simulink model "closedloopDAB"  (R2024b)
settings: Solver=ode23t  StartTime=0.0  StopTime=0.01  FixedStep=Tsolver  MaxStep=Tsolver  RelTol=1e-05
values from neighbouring files (symbols this model uses):
  D1 = M.D(k,1)    [closedloop_init.m]    (also in validate_exact_model.m)
  D2 = M.D(k,2)    [closedloop_init.m]    (also in validate_exact_model.m)
  D3 = M.D(k,3)    [closedloop_init.m]    (also in validate_exact_model.m)
  f_sw = P.fs    [closedloop_init.m]    (also in validate_exact_model.m)
  i2_cmd_max = umax_cmd    [closedloop_init.m]
  i2_cmd_min = -umax_cmd    [closedloop_init.m]
  Iref0 = -41.3    [closedloop_init.m]
  Iref1 = -46.3    [closedloop_init.m]
  ki_cmd = -5.2995    [closedloop_init.m]
  kp_cmd = -5.2995e-05    [closedloop_init.m]
  Ri = P.R1    [closedloop_init.m]    (also in validate_exact_model.m)
  Ro = P.R2    [closedloop_init.m]    (also in validate_exact_model.m)
  Rs = P.R    [closedloop_init.m]    (also in validate_exact_model.m)
  t_step = 5e-3    (= 0.005)    [closedloop_init.m]
  tdead = 0    [closedloop_init.m]    (also in validate_exact_model.m)
  umax_cmd = 0.8*min(D3 - 0, (D1 - D2) - D3)    [closedloop_init.m]
  Vi = P.V1    [closedloop_init.m]    (also in validate_exact_model.m)
  Vo = P.V2    [closedloop_init.m]    (also in validate_exact_model.m)
  Vth = 0.5    [closedloop_init.m]    (also in validate_exact_model.m)
libraries: fl_lib x15, nesl_utility x13, ee_lib x8, slpidlib x1, simulink x1
settings Model: Creator=amina  LastModifiedBy=amina
settings DataIOCC: SaveOutput=off  SignalLogging=off  DSMLogging=off  SaveTime=off  ReturnWorkspaceOutputs=off  ReturnWorkspaceOutputsName=out_fwd

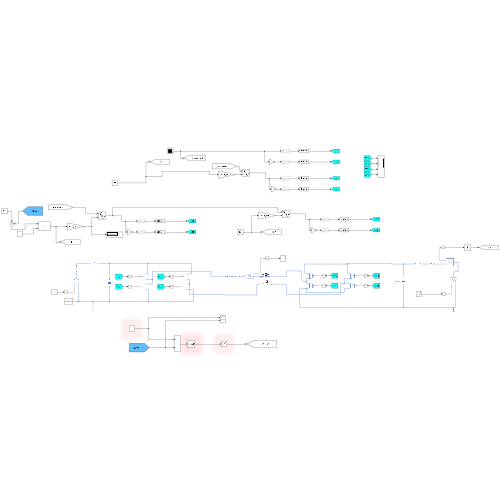
[thumbnail: Simulink's stored preview of the top-level diagram]
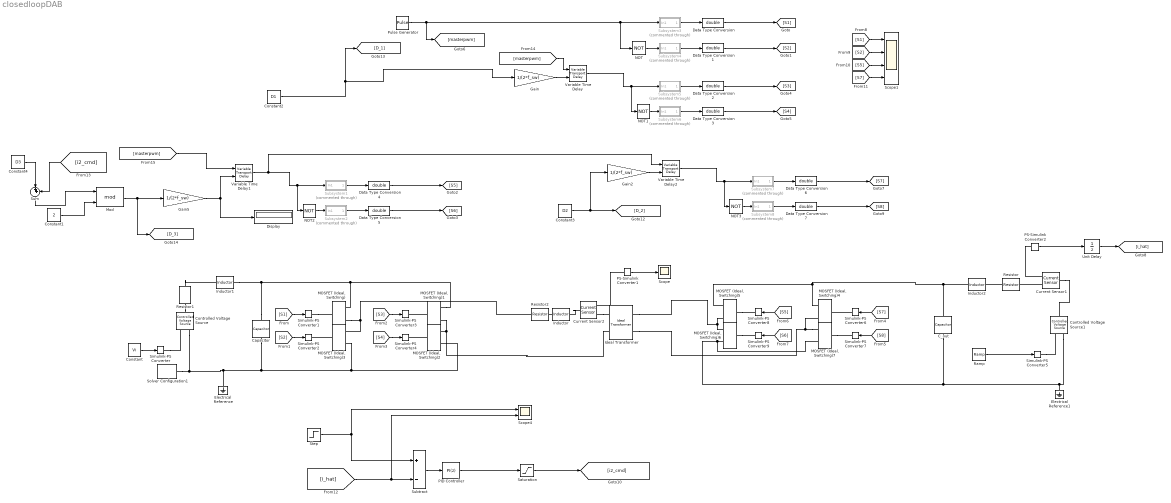
== system closedloopDAB ==
  C_out : fl_lib/Electrical/Electrical Elements/Capacitor  c=Co F  r=0 Ohm  g=0 1/Ohm  i_specify=off  i_priority=None  i=0 A  i_nominal_specify=off  i_nominal_value=1  i_nominal_unit=A  v_specify=off  v_priority=None  v=0 V  v_nominal_specify=off  v_nominal_value=1  v_nominal_unit=V  vc_specify=off  vc_priority=High  vc=V_cap_init V  vc_nominal_specify=off  vc_nominal_value=1  vc_nominal_unit=V
  Capacitor : fl_lib/Electrical/Electrical Elements/Capacitor  c=Ci F  r=1e-6 Ohm  g=0 1/Ohm  i_specify=off  i_priority=None  i=0 A  i_nominal_specify=off  i_nominal_value=1  i_nominal_unit=A  v_specify=off  v_priority=None  v=0 V  v_nominal_specify=off  v_nominal_value=1  v_nominal_unit=V  vc_specify=off  vc_priority=High  vc=V_cap_init V  vc_nominal_specify=off  vc_nominal_value=1  vc_nominal_unit=V
  Constant : Constant  Value=Vi
  Constant1 : Constant  Value=2
  Constant2 : Constant  Value=D1
  Constant3 : Constant  Value=D2
  Constant4 : Constant  Value=D3
  Controlled Voltage Source : fl_lib/Electrical/Electrical Sources/Controlled Voltage Source
  Controlled Voltage Source1 : fl_lib/Electrical/Electrical Sources/Controlled Voltage Source
  Current Sensor1 : fl_lib/Electrical/Electrical Sensors/Current Sensor
  Current Sensor2 : fl_lib/Electrical/Electrical Sensors/Current Sensor
  Data Type Conversion{,1..7} (8 alike) : DataTypeConversion  OutDataTypeStr=double  SaturateOnIntegerOverflow=off  RndMeth=Floor
  Display : Display
  Electrical Reference : fl_lib/Electrical/Electrical Elements/Electrical Reference
  Electrical Reference1 : fl_lib/Electrical/Electrical Elements/Electrical Reference
  Gain : Gain  Gain=1/(2*f_sw)
  Gain2 : Gain  Gain=1/(2*f_sw)
  Gain5 : Gain  Gain=1/(2*f_sw)
  Ideal Transformer : fl_lib/Electrical/Electrical Elements/Ideal Transformer  n=n  i1_specify=off  i1_priority=None  i1=0 A  i1_nominal_specify=off  i1_nominal_value=1  i1_nominal_unit=A  v1_specify=off  v1_priority=None  v1=0 V  v1_nominal_specify=off  v1_nominal_value=1  v1_nominal_unit=V  i2_specify=off  i2_priority=None  i2=0 A  i2_nominal_specify=off  i2_nominal_value=1  i2_nominal_unit=A  v2_specify=off  v2_priority=None  v2=0 V  v2_nominal_specify=off  v2_nominal_value=1  v2_nominal_unit=V
  Inductor : fl_lib/Electrical/Electrical Elements/Inductor  l=Ls H  r=0 Ohm  g=1e-9 1/Ohm  i_specify=off  i_priority=None  i=0 A  i_nominal_specify=off  i_nominal_value=1  i_nominal_unit=A  v_specify=off  v_priority=None  v=0 V  v_nominal_specify=off  v_nominal_value=1  v_nominal_unit=V  i_L_specify=off  i_L_priority=High  i_L=0 A  i_L_nominal_specify=off  i_L_nominal_value=1  i_L_nominal_unit=A
  Inductor1 : fl_lib/Electrical/Electrical Elements/Inductor  l=Li H  r=0 Ohm  g=1e-9 1/Ohm  i_specify=off  i_priority=None  i=0 A  i_nominal_specify=off  i_nominal_value=1  i_nominal_unit=A  v_specify=off  v_priority=None  v=0 V  v_nominal_specify=off  v_nominal_value=1  v_nominal_unit=V  i_L_specify=off  i_L_priority=High  i_L=0 A  i_L_nominal_specify=off  i_L_nominal_value=1  i_L_nominal_unit=A
  Inductor2 : fl_lib/Electrical/Electrical Elements/Inductor  l=Lo H  r=0 Ohm  g=1e-9 1/Ohm  i_specify=off  i_priority=None  i=0 A  i_nominal_specify=off  i_nominal_value=1  i_nominal_unit=A  v_specify=off  v_priority=None  v=0 V  v_nominal_specify=off  v_nominal_value=1  v_nominal_unit=V  i_L_specify=off  i_L_priority=High  i_L=0 A  i_L_nominal_specify=off  i_L_nominal_value=1  i_L_nominal_unit=A
  MOSFET (Ideal, Switching){,1..7} (8 alike) : ee_lib/Semiconductors & Converters/MOSFET (Ideal, Switching)  port_option=ee.enum.controlport.ps  Rds=Rds Ohm  Goff=G_mosfet 1/Ohm  Vth=Vth V  diode_param=ee.enum.semiconductors.protectionDiode.nodynamics  diode_Vf=0.8 V  diode_Ron=0.001 Ohm  diode_Goff=1e-5 1/Ohm  diode_C=50e-9 F  diode_iRM=-235 A  diode_iF=300 A  diode_idot=-50 A/us  diode_trr_param=ee.enum.converters.diodeReverseParam.trr_factor  diode_trr_factor=3  diode_trr=15 us  diode_Qrr=1500 s*uA  ids_specify=off  ids_priority=None  ids=0 A  ids_nominal_specify=off  ids_nominal_value=1  ids_nominal_unit=A  vds_specify=off  vds_priority=None  vds=0 V  vds_nominal_specify=off  vds_nominal_value=1  vds_nominal_unit=V  vgs_specify=off  vgs_priority=None  vgs=0 V  vgs_nominal_specify=off  vgs_nominal_value=1  vgs_nominal_unit=V  thermal_loss_option=ee.enum.converters.thermalLossOption.constantvalues  Von_data=[0, 1.8, 3.2, 6, 10, 16; 0, 2, 5.5, 9.5, 15, 25] V  Tj=[298.15, 448.15] K  Iout_data=[0, 20, 40, 60, 80, 100] A  Eon_data=[0, 55.04, 124.57, 235.53, 362.12; 0, 71.25, 161.25, 304.88, 468.75] * 1e-6 J  Eoff_data=[0, 18, 30, 56.1, 76.5; 0, 22.5, 37.5, 70.13, 95.63] * 1e-6 J  Eon_data_3D=[zeros(2, 5, 3)] J  Eoff_data_3D=[zeros(2, 5, 3)] J  Tj_loss=[298.15, 448.15] K  Iout_data_loss=[0, 10, 20, 30, 40] A  tabulateWithVds=false  Vds_loss=[0, 150, 300] V  Eon_scalar=22.86e-3 J  Eoff_scalar=17.14e-3 J  Voff=300 V  Iout_scalar=600 A  useCurrentFromPreviousCycle=false  useVoltageFromPreviousCycle=false  diodeModelType=ee.enum.converters.diodeModelType.pwl  diodeTableType=ee.enum.diode.tableType.IfMat  diode_ReverseIVType=ee.enum.diode.diodeReverseIV.constant  diode_IfMat=[.07, .12, .19, 1.75, 4.24, 7.32, 11.2; .16, .3, .72, 2.14, 4.02, 6.35, 9.12] A  diode_VfMat=[.9, 1.15, 1.25, 1.5, 1.75, 2.17, 2.6, 2.85; .58, .68, .75, 1.1, 1.38, 1.77, 2.27, 2.7] V  diode_TjVec=[25, 125] degC  diode_VfVec=[.5, .7, .9, 1.3, 1.7, 2.1, 2.5] V  diode_IfVec=[.1, .2, .5, 1, 2, 4, 7, 10] A  diode_IrMat=[1e-06, 2e-06, 5e-06, 1e-05, 2.5e-05, 5e-05, .0001; 2e-06, 5e-06, 1e-05, 4e-05, 8e-05, .0002, .0005] A  diode_VrMat=[10, 100, 200, 250, 300, 325, 350; 10, 70, 160, 220, 270, 300, 320] V  diode_VrVec=[10, 20, 40, 50, 70, 80, 100] V  diode_IrVec=[1e-06, 2e-06, 5e-06, 1e-05, 2e-05, 5e-05, .0001] A  diode_Vr=-600 V  diode_Ls=150 nH  diode_Erec=0.03 J  diode_rec_loss_model=ee.enum.diode.reverseRecoveryModel.fixed  diode_ErecVal=0 J  diode_scaleWithIandV=true  diode_ErecMat=zeros(2, 3) J  diode_TjrecVec=[298.15, 398.15] K  diode_IfrecVec=[.1, 1, 10] A  diode_IrecVal=10 A  diode_VrecVal=10 V  diode_tFilter=1 / 1000 / 100 s  separateThermalPortForDiode=false  thermal_network_parameterization=ee.enum.thermalNetworkTopology.external  Rth=[.03, .2] K/W  Rth_Cauer=[.03, .1, .2] K/W  Rth_Foster=[.08, .14, .22, .16] K/W  thermal_mass_parameterization=ee.enum.thermalNetwork.timeconstant  thermal_mass=[3, 25] J/K  thermal_mass_Cauer=[3, 10, 25] J/K  thermal_mass_Foster=[.001, .005, .05, .5] J/K  thermal_time_constant=[.1, 5] s  thermal_time_constant_Cauer=[.1, 1, 5] s  thermal_time_constant_Foster=[7e-05, .0007, .01, .08] s  thermal_mass_initial_temperatures=[25, 25] degC  thermal_mass_initial_temperatures_Cauer=[25, 25, 25] degC  junction_thermal_mass=0.1 J/K  Tvec_initial_Foster=[25, 25, 25, 25] degC  RthDiode=[.03, .2] K/W  RthCauerDiode=[.03, .1, .2] K/W  RthFosterDiode=[.03, .2] K/W  thermalMassDiode=[3, 25] J/K  thermalMassCauerDiode=[3, 10, 25] J/K  thermalMassFosterDiode=[33, 50] J/K  thermalTauDiode=[.1, 5] s  thermalTauCauerDiode=[.1, 1, 5] s  thermalTauFosterDiode=[1, 10] s  thermalMassInitTempDiode=[25, 25] degC  thermalMassInitTempCauerDiode=[25, 25, 25] degC  junctionthermalMassDiode=0.1 J/K  TVecInitialFosterDiode=[25, 25, 25, 25] degC  no_thermal_network=0  mosfet_junction_temperature_specify=off  mosfet_junction_temperature_priority=None  mosfet_junction_temperature=25 degC  mosfet_junction_temperature_nominal_specify=off  mosfet_junction_temperature_nominal_value=1  mosfet_junction_temperature_nominal_unit=degC  diode_junction_temperature_specify=off  diode_junction_temperature_priority=None  diode_junction_temperature=25 degC  diode_junction_temperature_nominal_specify=off  diode_junction_temperature_nominal_value=1  diode_junction_temperature_nominal_unit=degC  Qj_specify=off  Qj_priority=None  Qj=0 W  Qj_nominal_specify=off  Qj_nominal_value=1  Qj_nominal_unit=W  accumulatedSwitchingLosses_specify=off  accumulatedSwitchingLosses_priority=None  accumulatedSwitchingLosses=0 J
  Mod : Math  Operator=mod
  NOT{,1..3} (4 alike) : Logic  Operator=NOT  IconShape=distinctive  AllPortsSameDT=off  OutDataTypeStr=boolean
  PID Controller : slpidlib/PID Controller  Controller=PI  Form=Parallel  TimeDomain=Discrete-time  UseExternalTs=off  SampleTime=1/f_sw  IntegratorMethod=Forward Euler  FilterMethod=Forward Euler  ControllerParametersSource=internal  P=kp_cmd  I=ki_cmd  UseKiTs=off  D=0  UseExternalDerivativeSource=off  N=100  UseFilter=on  TunerSelectOption=Transfer Function Based (PID Tuner App)  InitialConditionSource=internal  InitialConditionForIntegrator=0  InitialConditionForFilter=0  DifferentiatorICPrevScaledInput=0  ExternalReset=none  TrackingMode=off  Kt=1  LimitOutput=on  SatLimitsSource=internal  UpperSaturationLimit=umax_cmd  LowerSaturationLimit=-umax_cmd  LinearizeAsGain=on  AntiWindupMode=clamping  Kb=1  LimitIntegrator=off  UpperIntegratorSaturationLimit=180  LowerIntegratorSaturationLimit=0  POutMin=[]  POutMax=[]  IOutMin=[]  IOutMax=[]  DOutMin=[]  DOutMax=[]  NOutMin=[]  NOutMax=[]  SumOutMin=[]  SumOutMax=[]  SaturationOutMin=[]  SaturationOutMax=[]  PParamMin=[]  PParamMax=[]  IParamMin=[]  IParamMax=[]  DParamMin=[]  DParamMax=[]  NParamMin=[]  NParamMax=[]  KbParamMin=[]  KbParamMax=[]  KtParamMin=[]  KtParamMax=[]  KbOutMin=[]  KbOutMax=[]  KtOutMin=[]  KtOutMax=[]  IntegratorOutMin=[]  IntegratorOutMax=[]  FilterOutMin=[]  FilterOutMax=[]  SumI1OutMin=[]  SumI1OutMax=[]  SumI2OutMin=[]  SumI2OutMax=[]  SumI3OutMin=[]  SumI3OutMax=[]  SumI4OutMin=[]  SumI4OutMax=[]  SumDOutMin=[]  SumDOutMax=[]  DifferentiatorOutMin=[]  DifferentiatorOutMax=[]  FilterDiffOutCoefMin=[]  FilterDiffOutCoefMax=[]  ReciprocalOutMin=[]  ReciprocalOutMax=[]  SumDenOutMin=[]  SumDenOutMax=[]  SumNumOutMin=[]  SumNumOutMax=[]  DivideOutMin=[]  DivideOutMax=[]  UdiffTsProdOutMin=[]  UdiffTsProdOutMax=[]  NTsProdOutMin=[]  NTsProdOutMax=[]  UintegralTsProdOutMin=[]  UintegralTsProdOutMax=[]  UngainTsProdOutMin=[]  UngainTsProdOutMax=[]  ClampingZeroOutDataTypeStr=Inherit: Inherit via back propagation  ClampingZeroOutMin=[]  ClampingZeroOutMax=[]  FilterDenConstantOutDataTypeStr=Inherit: Inherit via back propagation  FilterDenConstantOutMin=[]  FilterDenConstantOutMax=[]  PCopyOutDataTypeStr=Inherit: Inherit via back propagation  PCopyOutMin=[]  PCopyOutMax=[]  NCopyOutDataTypeStr=Inherit: Inherit via back propagation  NCopyOutMin=[]  NCopyOutMax=[]  IntegratorContinuousStateAttributes=''  IntegratorStateMustResolveToSignalObject=off  IntegratorRTWStateStorageClass=Auto  FilterContinuousStateAttributes=''  FilterStateMustResolveToSignalObject=off  FilterRTWStateStorageClass=Auto  ParallelPVariant=InternalParameters  IdealPVariant=Disabled  IVariant=InternalParameters  DVariant=Disabled  IntegratorVariant=Discrete  SatVariant=Enabled  AWVariant=DiscClampingParallel  PCopyVariant=Disabled  TRVariant=Disabled  FdbkBlocksVariant=Forward  IdealPFdbkVariant=Disabled  SatFdbkVariant=Disabled  DerivativeFilterVariant=Disabled  NVariant=Disabled  NCopyVariant=Disabled_SignalSpec  FilterICVariant=Disabled  IntegratorICVariant=InternalICs  ExternalResetVariant=Disabled  TRSumVariant=Passthrough  SumFdbkVariant=Disabled  SumVariant=Sum_PI  TsampFilterVariant=InternalTs  TsampNgainVariant=Passthrough  TsampIntegralVariant=Disabled_SignalSpec  ExternalSaturationOutDataTypeStr=Inherit: Same as second input  DerivativeSourceVariant=Disabled  PreIntVariant=InternalPreInt
  PS-Simulink Converter1 : nesl_utility/PS-Simulink Converter  PhysicalDomain=network_engine_domain  SubClassName=ps_output  LeftPortType=input  RightPortType=output  PseudoPeriodic=off  Frequencies=[]  VectorFormat=inherit  Unit=inherit  AffineConversion=off
  PS-Simulink Converter2 : nesl_utility/PS-Simulink Converter  PhysicalDomain=network_engine_domain  SubClassName=ps_output  LeftPortType=input  RightPortType=output  PseudoPeriodic=off  Frequencies=[]  VectorFormat=inherit  Unit=inherit  AffineConversion=off
  Pulse Generator : DiscretePulseGenerator  PulseType=Time based  Period=1/f_sw  PulseWidth=50
  Ramp : simulink/Sources/Ramp  slope=0  start=0  InitialOutput=Vo
  Resistor : fl_lib/Electrical/Electrical Elements/Resistor  R=Ro Ohm  i_specify=off  i_priority=None  i=0 A  i_nominal_specify=off  i_nominal_value=1  i_nominal_unit=A  v_specify=off  v_priority=None  v=0 V  v_nominal_specify=off  v_nominal_value=1  v_nominal_unit=V
  Resistor1 : fl_lib/Electrical/Electrical Elements/Resistor  R=Ri Ohm  i_specify=off  i_priority=None  i=0 A  i_nominal_specify=off  i_nominal_value=1  i_nominal_unit=A  v_specify=off  v_priority=None  v=0 V  v_nominal_specify=off  v_nominal_value=1  v_nominal_unit=V
  Resistor2 : fl_lib/Electrical/Electrical Elements/Resistor  R=Rs Ohm  i_specify=off  i_priority=None  i=0 A  i_nominal_specify=off  i_nominal_value=1  i_nominal_unit=A  v_specify=off  v_priority=None  v=0 V  v_nominal_specify=off  v_nominal_value=1  v_nominal_unit=V
  Saturation : Saturate  UpperLimit=i2_cmd_max  LowerLimit=i2_cmd_min
  Scope : Scope
  Scope1 : Scope  NumInputPorts=4
  Scope4 : Scope  NumInputPorts=2
  Simulink-PS Converter{,1..9} (10 alike) : nesl_utility/Simulink-PS Converter  PhysicalDomain=network_engine_domain  SubClassName=ps_input  LeftPortType=input  RightPortType=output  PseudoPeriodic=off  Frequencies=[]  NoiseDistribution=none  NoiseParameters=[]  Unit=1  AffineConversion=off  FilteringAndDerivatives=provide  SimscapeFilterOrder=1  InputFilterTimeConstant=0.001  UdotUserProvided=0
  Solver Configuration1 : nesl_utility/Solver Configuration  PhysicalDomain=network_engine_domain  SubClassName=solver  LeftPortType=input  RightPortType=generic  Tones=[]  Harmonics=[]  SimulateNoise=off  Profile=off  UseLocalSampling=off  EnableSwitchedLinearOptims=on  FrequencyDomain=off  UseCCode=off  RelTol=0.001  AbsTol=1e-06  MinStep=1e-09  ToWorkspace=off  RevertToSquareIcSolve=off  NumHomotopyIterations=100  PhasorMode=off  PhasorModeNumHarmonics=1  ConsistencySolver=NEWTON_FTOL  IndexReductionMethod=DerivativeReplacement  DoDC=off  ResidualTolerance=1e-09  ConsistencyTolSource=GLOBAL  ConsistencyAbsTol=0.001  ConsistencyRelTol=0.001  ConsistencyTolFactor=0.001  UseLocalSolver=off  LocalSolverChoice=NE_BACKWARD_EULER_ADVANCER  ResolveIndetEquations=on  FunctionEvalNumThread=1  LocalSolverSampleTime=0.001  DoFixedCost=off  MaxNonlinIter=3  MaxModeIter=2  ComputeImpulses=off  ImpulseIterations=2  LinearAlgebra=auto  LinearAlgebraNumThread=0  EquationFormulation=NE_TIME_EF  DelaysMemoryBudget=1024  AutomaticFiltering=on  FilteringTimeConstant=0.001  PartitionStorageMethod=AS_NEEDED  PartitionMemoryBudget=1024  PartitionMethod=ROBUST  MultibodyUseLocalSolver=off  MultibodyLocalSolverChoice=ODE1  MultibodyLocalSolverSampleTime=0.001
  Step : Step  Time=t_step  Before=Iref0  After=Iref1  SampleTime=0
  Subsystem1 : Subsystem  Commented=through
  Subsystem2 : Subsystem  Commented=through
  Subsystem3 : Subsystem  Commented=through
  Subsystem4 : Subsystem  Commented=through
  Subsystem5 : Subsystem  Commented=through
  Subsystem6 : Subsystem  Commented=through
  Subsystem7 : Subsystem  Commented=through
  Subsystem8 : Subsystem  Commented=through
  Subtract : Sum  Inputs=+-
  Sum : Sum  Inputs=|++
  Unit Delay : UnitDelay  SampleTime=1/f_sw  HasFrameUpgradeWarning=on
  Variable Time Delay : VariableTransportDelay  MaximumDelay=10
  Variable Time Delay1 : VariableTransportDelay  MaximumDelay=10
  Variable Time Delay2 : VariableTransportDelay  MaximumDelay=10
  wires:
  Gain/1 -> Variable Time Delay/2
  Subsystem6/1(Out1) -> Data Type Conversion3/1
  Subsystem8/1(Out1) -> Data Type Conversion7/1
  Subsystem7/1(Out1) -> Data Type Conversion6/1
  Pulse Generator/1 -> [masterpwm], Subsystem3/1(In1), NOT/1
  [masterpwm] -> Variable Time Delay1/1
  NOT1/1 -> Subsystem6/1(In1)
  Data Type Conversion/1 -> [S1]
  Subsystem1/1(Out1) -> Data Type Conversion4/1
  NOT/1 -> Subsystem4/1(In1)
  Constant/1 -> Simulink-PS Converter/1
  [S1] -> Scope1/1
  Subsystem2/1(Out1) -> Data Type Conversion5/1
  Variable Time Delay1/1 -> Variable Time Delay2/1, NOT2/1, Subsystem1/1(In1)
  [S2] -> Scope1/2
  [S3] -> Simulink-PS Converter3/1
  [S4] -> Simulink-PS Converter4/1
  [S1] -> Simulink-PS Converter1/1
  [masterpwm] -> Variable Time Delay/1
  Variable Time Delay/1 -> NOT1/1, Subsystem5/1(In1)
  Subsystem5/1(Out1) -> Data Type Conversion2/1
  Variable Time Delay2/1 -> NOT3/1, Subsystem7/1(In1)
  [S6] -> Simulink-PS Converter9/1
  [S7] -> Scope1/4
  [S7] -> Simulink-PS Converter6/1
  Gain5/1 -> Display/1, Variable Time Delay1/2
  NOT2/1 -> Subsystem2/1(In1)
  Data Type Conversion6/1 -> [S7]
  Data Type Conversion4/1 -> [S5]
  Data Type Conversion1/1 -> [S2]
  Data Type Conversion7/1 -> [S8]
  Data Type Conversion5/1 -> [S6]
  [S5] -> Scope1/3
  Data Type Conversion3/1 -> [S4]
  Gain2/1 -> Variable Time Delay2/2
  Constant1/1 -> Mod/2
  [S2] -> Simulink-PS Converter2/1
  Data Type Conversion2/1 -> [S3]
  Mod/1 -> [D_3], Gain5/1
  NOT3/1 -> Subsystem8/1(In1)
  PS-Simulink Converter1/1 -> Scope/1
  [S5] -> Simulink-PS Converter8/1
  [S8] -> Simulink-PS Converter7/1
  Subsystem3/1(Out1) -> Data Type Conversion/1
  Subsystem4/1(Out1) -> Data Type Conversion1/1
  Step/1 -> Subtract/1, Scope4/1
  Subtract/1 -> PID Controller/1
  Unit Delay/1 -> [i_hat]
  PS-Simulink Converter2/1 -> Unit Delay/1
  Saturation/1 -> [i2_cmd]
  Constant3/1 -> [D_2], Gain2/1
  Constant2/1 -> Gain/1, [D_1]
  [i_hat] -> Subtract/2, Scope4/2
  Ramp/1 -> Simulink-PS Converter5/1
  Constant4/1 -> Sum/1
  [i2_cmd] -> Sum/2
  Sum/1 -> Mod/1
  PID Controller/1 -> Saturation/1
  connections:
  Controlled Voltage Source/RConn2 -- Solver Configuration1/RConn1 -- Electrical Reference/LConn1 -- "MOSFET (Ideal, Switching)2"/RConn2 -- "MOSFET (Ideal, Switching)3"/RConn2 -- Capacitor/RConn1
  Capacitor/LConn1 -- "MOSFET (Ideal, Switching)1"/RConn1 -- "MOSFET (Ideal, Switching)"/RConn1 -- Inductor1/RConn1
  C_out/RConn1 -- Controlled Voltage Source1/RConn2 -- Electrical Reference1/LConn1 -- "MOSFET (Ideal, Switching)6"/RConn2 -- "MOSFET (Ideal, Switching)7"/RConn2
  Resistor2/RConn1 -- "MOSFET (Ideal, Switching)3"/RConn1 -- "MOSFET (Ideal, Switching)"/RConn2
  "MOSFET (Ideal, Switching)1"/RConn2 -- Ideal Transformer/LConn2 -- "MOSFET (Ideal, Switching)2"/RConn1
  Inductor2/LConn1 -- C_out/LConn1 -- "MOSFET (Ideal, Switching)4"/RConn1 -- "MOSFET (Ideal, Switching)5"/RConn1
  "MOSFET (Ideal, Switching)5"/RConn2 -- Ideal Transformer/RConn1 -- "MOSFET (Ideal, Switching)6"/RConn1
  "MOSFET (Ideal, Switching)7"/RConn1 -- Ideal Transformer/RConn2 -- "MOSFET (Ideal, Switching)4"/RConn2
  Simulink-PS Converter5/RConn1 -- Controlled Voltage Source1/RConn1
  Simulink-PS Converter6/RConn1 -- "MOSFET (Ideal, Switching)4"/LConn1
  Current Sensor2/LConn1 -- Inductor/RConn1
  Simulink-PS Converter/RConn1 -- Controlled Voltage Source/RConn1
  Resistor2/LConn1 -- Inductor/LConn1
  Resistor1/RConn1 -- Controlled Voltage Source/LConn1
  PS-Simulink Converter1/LConn1 -- Current Sensor2/RConn1
  "MOSFET (Ideal, Switching)6"/LConn1 -- Simulink-PS Converter9/RConn1
  "MOSFET (Ideal, Switching)1"/LConn1 -- Simulink-PS Converter3/RConn1
  Current Sensor2/RConn2 -- Ideal Transformer/LConn1
  "MOSFET (Ideal, Switching)3"/LConn1 -- Simulink-PS Converter2/RConn1
  "MOSFET (Ideal, Switching)2"/LConn1 -- Simulink-PS Converter4/RConn1
  "MOSFET (Ideal, Switching)7"/LConn1 -- Simulink-PS Converter7/RConn1
  Simulink-PS Converter1/RConn1 -- "MOSFET (Ideal, Switching)"/LConn1
  Resistor1/LConn1 -- Inductor1/LConn1
  "MOSFET (Ideal, Switching)5"/LConn1 -- Simulink-PS Converter8/RConn1
  Resistor/RConn1 -- Inductor2/RConn1
  Current Sensor1/RConn2 -- Resistor/LConn1
  Current Sensor1/LConn1 -- Controlled Voltage Source1/LConn1
  Current Sensor1/RConn1 -- PS-Simulink Converter2/LConn1

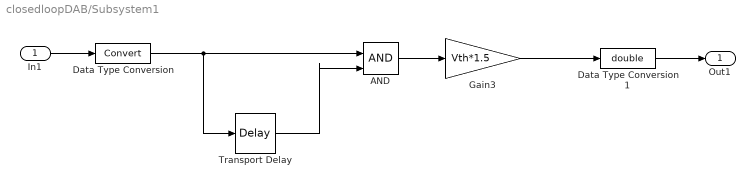
== system closedloopDAB/Subsystem1 ==
  In1 : Inport
  AND : Logic  IconShape=distinctive  AllPortsSameDT=off  OutDataTypeStr=boolean
  Data Type Conversion : DataTypeConversion  SaturateOnIntegerOverflow=off  RndMeth=Floor
  Data Type Conversion1 : DataTypeConversion  OutDataTypeStr=double  SaturateOnIntegerOverflow=off  RndMeth=Floor
  Gain3 : Gain  Gain=Vth*1.5
  Transport Delay : TransportDelay  DelayTime=tdead
  Out1 : Outport
  wires:
  Data Type Conversion/1 -> AND/1, Transport Delay/1
  In1/1 -> Data Type Conversion/1
  Transport Delay/1 -> AND/2
  AND/1 -> Gain3/1
  Gain3/1 -> Data Type Conversion1/1
  Data Type Conversion1/1 -> Out1/1

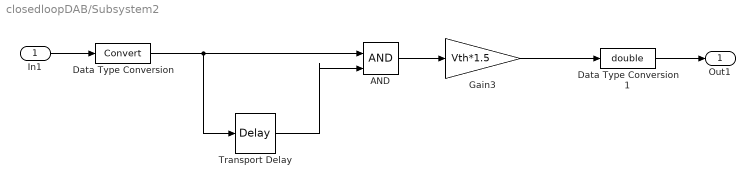
== system closedloopDAB/Subsystem2 ==
  In1 : Inport
  AND : Logic  IconShape=distinctive  AllPortsSameDT=off  OutDataTypeStr=boolean
  Data Type Conversion : DataTypeConversion  SaturateOnIntegerOverflow=off  RndMeth=Floor
  Data Type Conversion1 : DataTypeConversion  OutDataTypeStr=double  SaturateOnIntegerOverflow=off  RndMeth=Floor
  Gain3 : Gain  Gain=Vth*1.5
  Transport Delay : TransportDelay  DelayTime=tdead
  Out1 : Outport
  wires:
  Data Type Conversion1/1 -> Out1/1
  Gain3/1 -> Data Type Conversion1/1
  AND/1 -> Gain3/1
  Transport Delay/1 -> AND/2
  In1/1 -> Data Type Conversion/1
  Data Type Conversion/1 -> Transport Delay/1, AND/1

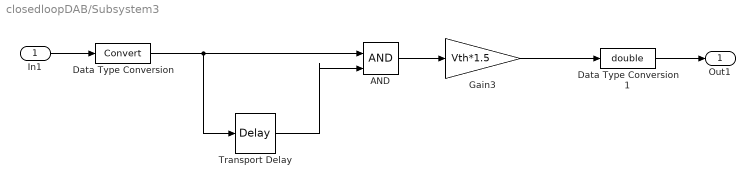
== system closedloopDAB/Subsystem3 ==
  In1 : Inport
  AND : Logic  IconShape=distinctive  AllPortsSameDT=off  OutDataTypeStr=boolean
  Data Type Conversion : DataTypeConversion  SaturateOnIntegerOverflow=off  RndMeth=Floor
  Data Type Conversion1 : DataTypeConversion  OutDataTypeStr=double  SaturateOnIntegerOverflow=off  RndMeth=Floor
  Gain3 : Gain  Gain=Vth*1.5
  Transport Delay : TransportDelay  DelayTime=tdead
  Out1 : Outport
  wires:
  Data Type Conversion/1 -> AND/1, Transport Delay/1
  In1/1 -> Data Type Conversion/1
  Transport Delay/1 -> AND/2
  AND/1 -> Gain3/1
  Gain3/1 -> Data Type Conversion1/1
  Data Type Conversion1/1 -> Out1/1

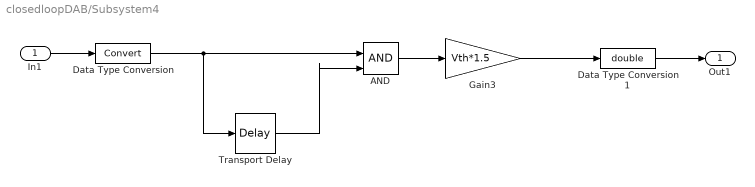
== system closedloopDAB/Subsystem4 ==
  In1 : Inport
  AND : Logic  IconShape=distinctive  AllPortsSameDT=off  OutDataTypeStr=boolean
  Data Type Conversion : DataTypeConversion  SaturateOnIntegerOverflow=off  RndMeth=Floor
  Data Type Conversion1 : DataTypeConversion  OutDataTypeStr=double  SaturateOnIntegerOverflow=off  RndMeth=Floor
  Gain3 : Gain  Gain=Vth*1.5
  Transport Delay : TransportDelay  DelayTime=tdead
  Out1 : Outport
  wires:
  Data Type Conversion1/1 -> Out1/1
  Gain3/1 -> Data Type Conversion1/1
  AND/1 -> Gain3/1
  Transport Delay/1 -> AND/2
  In1/1 -> Data Type Conversion/1
  Data Type Conversion/1 -> Transport Delay/1, AND/1

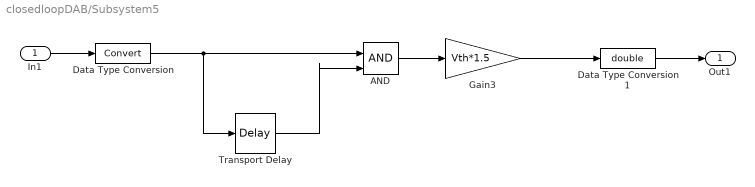
== system closedloopDAB/Subsystem5 ==
  In1 : Inport
  AND : Logic  IconShape=distinctive  AllPortsSameDT=off  OutDataTypeStr=boolean
  Data Type Conversion : DataTypeConversion  SaturateOnIntegerOverflow=off  RndMeth=Floor
  Data Type Conversion1 : DataTypeConversion  OutDataTypeStr=double  SaturateOnIntegerOverflow=off  RndMeth=Floor
  Gain3 : Gain  Gain=Vth*1.5
  Transport Delay : TransportDelay  DelayTime=tdead
  Out1 : Outport
  wires:
  Data Type Conversion/1 -> AND/1, Transport Delay/1
  In1/1 -> Data Type Conversion/1
  Transport Delay/1 -> AND/2
  AND/1 -> Gain3/1
  Gain3/1 -> Data Type Conversion1/1
  Data Type Conversion1/1 -> Out1/1

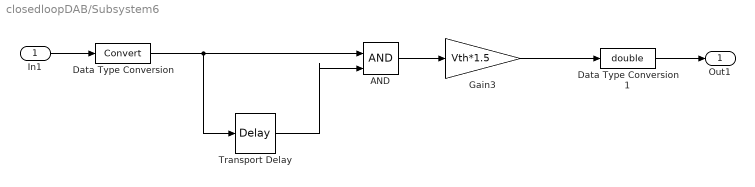
== system closedloopDAB/Subsystem6 ==
  In1 : Inport
  AND : Logic  IconShape=distinctive  AllPortsSameDT=off  OutDataTypeStr=boolean
  Data Type Conversion : DataTypeConversion  SaturateOnIntegerOverflow=off  RndMeth=Floor
  Data Type Conversion1 : DataTypeConversion  OutDataTypeStr=double  SaturateOnIntegerOverflow=off  RndMeth=Floor
  Gain3 : Gain  Gain=Vth*1.5
  Transport Delay : TransportDelay  DelayTime=tdead
  Out1 : Outport
  wires:
  Data Type Conversion1/1 -> Out1/1
  Gain3/1 -> Data Type Conversion1/1
  AND/1 -> Gain3/1
  Transport Delay/1 -> AND/2
  In1/1 -> Data Type Conversion/1
  Data Type Conversion/1 -> Transport Delay/1, AND/1

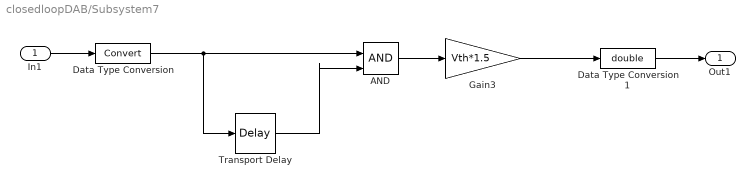
== system closedloopDAB/Subsystem7 ==
  In1 : Inport
  AND : Logic  IconShape=distinctive  AllPortsSameDT=off  OutDataTypeStr=boolean
  Data Type Conversion : DataTypeConversion  SaturateOnIntegerOverflow=off  RndMeth=Floor
  Data Type Conversion1 : DataTypeConversion  OutDataTypeStr=double  SaturateOnIntegerOverflow=off  RndMeth=Floor
  Gain3 : Gain  Gain=Vth*1.5
  Transport Delay : TransportDelay  DelayTime=tdead
  Out1 : Outport
  wires:
  Data Type Conversion/1 -> AND/1, Transport Delay/1
  In1/1 -> Data Type Conversion/1
  Transport Delay/1 -> AND/2
  AND/1 -> Gain3/1
  Gain3/1 -> Data Type Conversion1/1
  Data Type Conversion1/1 -> Out1/1

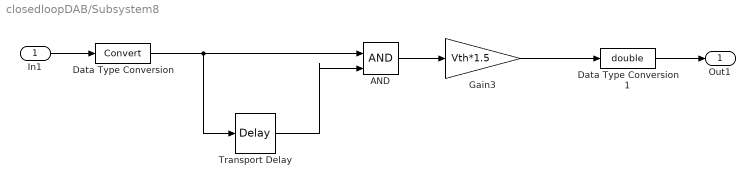
== system closedloopDAB/Subsystem8 ==
  In1 : Inport
  AND : Logic  IconShape=distinctive  AllPortsSameDT=off  OutDataTypeStr=boolean
  Data Type Conversion : DataTypeConversion  SaturateOnIntegerOverflow=off  RndMeth=Floor
  Data Type Conversion1 : DataTypeConversion  OutDataTypeStr=double  SaturateOnIntegerOverflow=off  RndMeth=Floor
  Gain3 : Gain  Gain=Vth*1.5
  Transport Delay : TransportDelay  DelayTime=tdead
  Out1 : Outport
  wires:
  Data Type Conversion1/1 -> Out1/1
  Gain3/1 -> Data Type Conversion1/1
  AND/1 -> Gain3/1
  Transport Delay/1 -> AND/2
  In1/1 -> Data Type Conversion/1
  Data Type Conversion/1 -> Transport Delay/1, AND/1
